simulink model "aero2_mechanical_linearization_experiment_R2021a"  (R2021a)
settings: Solver=ode1  StartTime=0.0  StopTime=2  FixedStep=0.002  RelTol=1e-3
model workspace (MAT data in the model file):
  X0 = [0.1; 0.2; -0.05; 0.04]
settings Model: Creator=matiasgarcia  LastModifiedBy=matiasgarcia
settings DataIOCC: SaveOutput=off  SignalLogging=off  SaveTime=off
settings DebuggingCC: UnconnectedInputMsg=none  UnconnectedOutputMsg=none  UnconnectedLineMsg=none
settings ModelReferenceCC: EnableRefExpFcnMdlSchedulingChecks=off
settings RTWCC: Description=Generic Real-Time Target  GPUComputeCapability=5.0  DLArmComputeVersion=20.02.1

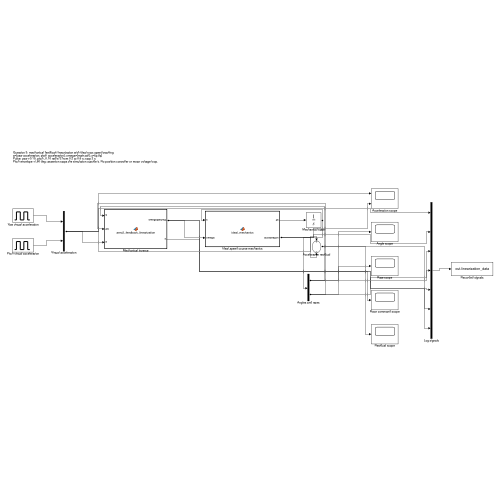
[thumbnail: Simulink's stored preview of the top-level diagram]
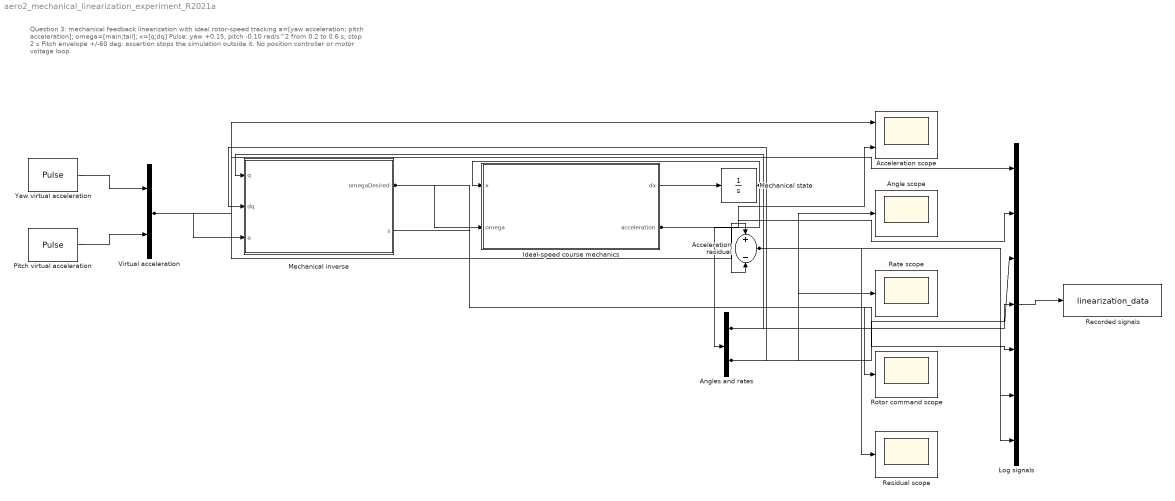
== system aero2_mechanical_linearization_experiment_R2021a ==
  note: Question 3: mechanical feedback linearization with ideal rotor-speed tracking
      | a=[yaw acceleration; pitch acceleration]; omega=[main;tail]; x=[q;dq]
      | Pulse: yaw +0.15, pitch -0.10 rad/s^2 from 0.2 to 0.6 s; stop 2 s
      | Pitch envelope +/-60 deg: assertion stops the simulation outside it. No position controller or motor voltage loop.
  Acceleration residual : Sum  Inputs=+-
  Acceleration scope : Scope  NumInputPorts=2
  Angle scope : Scope
  Angles and rates : Demux  Outputs=[2 2]
  Ideal-speed course mechanics : MATLAB Function  TreatAsAtomicUnit=on
  Log signals : Mux  Inputs=7
  Mechanical inverse : MATLAB Function  TreatAsAtomicUnit=on
  Mechanical state : Integrator  InitialCondition=X0
  Pitch virtual acceleration : DiscretePulseGenerator  PulseType=Time based  Amplitude=-0.1  Period=10  PulseWidth=4  PhaseDelay=0.2  SampleTime=0
  Rate scope : Scope
  Recorded signals : ToWorkspace  VariableName=linearization_data  SaveFormat=Timeseries  SampleTime=-1
  Residual scope : Scope
  Rotor command scope : Scope
  Virtual acceleration : Mux  Inputs=2
  Yaw virtual acceleration : DiscretePulseGenerator  PulseType=Time based  Amplitude=0.15  Period=10  PulseWidth=4  PhaseDelay=0.2  SampleTime=0
  wires:
  Yaw virtual acceleration/1 -> Virtual acceleration/1
  Pitch virtual acceleration/1 -> Virtual acceleration/2
  Virtual acceleration/1 -> Mechanical inverse/3(a), Acceleration residual/1, Acceleration scope/1, Log signals/1
  Mechanical inverse/1(omegaDesired) -> Ideal-speed course mechanics/2(omega), Rotor command scope/1, Log signals/5
  Ideal-speed course mechanics/1(dx) -> Mechanical state/1
  Mechanical state/1 -> Ideal-speed course mechanics/1(x), Angles and rates/1
  Angles and rates/1 -> Mechanical inverse/1(q), Angle scope/1, Log signals/3
  Angles and rates/2 -> Mechanical inverse/2(dq), Rate scope/1, Log signals/4
  Ideal-speed course mechanics/2(acceleration) -> Acceleration residual/2, Acceleration scope/2, Log signals/2
  Acceleration residual/1 -> Residual scope/1, Log signals/7
  Mechanical inverse/2(s) -> Log signals/6
  Log signals/1 -> Recorded signals/1

== matlab function aero2_mechanical_linearization_experiment_R2021a/Ideal-speed course mechanics ==
  data: x input; dx output; omega input; acceleration output
function [dx, acceleration] = ideal_mechanics(x, omega)
fullDerivative = course_dynamics([0;0], [x;omega]);
dx = fullDerivative(1:4);
acceleration = fullDerivative(3:4);
end

function dx = course_dynamics(u, x)
%% Simplified twin-rotor model of aero2_model.pdf (2-DOF body + first-order motors)
p = struct('Jph', 0.64070000000000005, ...
    'jph', 0.01, ...
    'Jth', 0.71640000000000004, ...
    'G', 0.025399999999999999, ...
    'kT', 4.2486999999999997e-06, ...
    'kF', 2.5525999999999999e-05, ...
    'L', 0.16700000000000001, ...
    'Cor', 0.63070000000000004, ...
    'Dph', 0, ...
    'Dth', 0, ...
    'aw', 5.7800000000000002, ...
    'bw', 96.531999999999996);
dx = tr_simp_dyn(x, u, p);
end

function dx = tr_simp_dyn(x, u, p)
%TR_SIMP_DYN  Simplified twin-rotor model with voltage inputs (aero2_model.pdf).
%   Body: reduced 2-DOF model, eq. (simp)
%     Mq(th) [ddpsi; ddth] + cq + Bq dq + gq = Gamma(th) [wm|wm|; wt|wt|]
%   with cq = [-Cor sin(2th) dth dpsi; 1/2 Cor sin(2th) dpsi^2]
%   (no gyroscopic coupling, no motor reaction channel, s_m=+1, s_t=-1).
%   Rotors: first-order motor model of the hand-out
%     dw = -aw w + bw v
%   State x = [psi, theta, dpsi, dtheta, wm, wt], input u = [Um, Ut].
%   p: Jph jph Jth Dph Dth Cor L G kF kT aw bw (psim of tr_instructor_params).

    th = x(2);  dps = x(3);  dth = x(4);
    c = cos(th);  s = sin(th);
    tau = [x(5)*abs(x(5)); x(6)*abs(x(6))];

    Ms  = [p.Jph*c^2 + p.jph*s^2, 0; 0, p.Jth];
    Cs  = [-p.Cor*sin(2*th)*dth*dps; 0.5*p.Cor*sin(2*th)*dps^2];
    Ds  = [p.Dph*dps; p.Dth*dth];
    Gs  = [0; p.G*s];
    Gam = [c 0; 0 1]*[-p.kT, p.L*p.kF; p.L*p.kF, p.kT];
    ddq = Ms\(Gam*tau - Cs - Ds - Gs);

    dw  = -p.aw*x(5:6) + p.bw*u(:);
    dx  = [x(3:4); ddq; dw];
end

== matlab function aero2_mechanical_linearization_experiment_R2021a/Mechanical inverse ==
  data: q input; omegaDesired output; dq input; a input; s output
function [omegaDesired, s] = aero2_feedback_linearization(q, dq, a)
%AERO2_FEEDBACK_LINEARIZATION Ideal motor tracking: choose omega for q_ddot=a.
% The signed square root is defined at zero but has no finite derivative there.
p = aero2_mechanical_parameters;
assert(abs(q(2)) <= p.pitchLimit, 'Pitch envelope exceeded (limit 60 deg).');
[M, c, g, Gamma] = aero2_mechanical_terms(q, dq);
s = Gamma\(M*a+c+g);
omegaDesired = sign(s).*sqrt(abs(s));
end

function [M, c, g, Gamma] = aero2_mechanical_terms(q, dq)
%AERO2_MECHANICAL_TERMS M*q_ddot+c+g=Gamma*(omega.*abs(omega)).
% Signal order: q=[yaw;pitch], dq=[yaw rate;pitch rate], omega=[main;tail].
p = aero2_mechanical_parameters;
theta = q(2);
cor = p.Jyaw-p.jyaw;
M = [p.Jyaw*cos(theta)^2+p.jyaw*sin(theta)^2, 0; 0, p.Jpitch];
c = [-cor*sin(2*theta)*dq(2)*dq(1); ...
    0.5*cor*sin(2*theta)*dq(1)^2];
g = [0; p.gravity*sin(theta)];
Gamma = [cos(theta), 0; 0, 1]*[-p.kt, p.lever*p.kf; p.lever*p.kf, p.kt];
end

function p = aero2_mechanical_parameters
%AERO2_MECHANICAL_PARAMETERS Simplified course model, Part II, pages 4-5.
p.Jyaw = 0.6407;
p.jyaw = 0.01;
p.Jpitch = 0.7164;
p.gravity = 0.0254;
p.kt = 4.2487e-6;
p.kf = 2.5526e-5;
p.lever = 0.167;
p.pitchLimit = pi/3; % Simulation envelope, not an approved hardware limit.
p.initialState = [0.1; 0.2; -0.05; 0.04]; % [yaw; pitch; yaw rate; pitch rate].
p.acceleration = [0.15; -0.1];
p.step = 0.002;
end
